simulink model "Task8_PWMSignal_2024b"  (R2025a)
settings: Solver=VariableStepAuto  StartTime=0.0  StopTime=10.0  RelTol=1e-3
libraries: simulink x2
settings Model: LastModifiedBy=Ashwin VJ

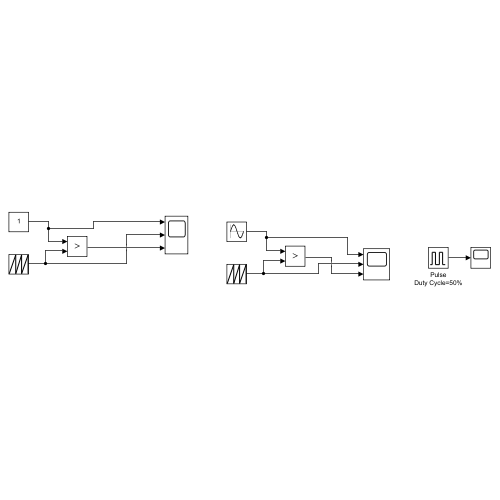
[thumbnail: Simulink's stored preview of the top-level diagram]
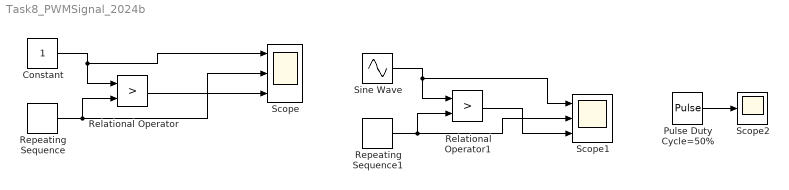
== system Task8_PWMSignal_2024b ==
  Constant : Constant
  Pulse Duty Cycle=50% : DiscretePulseGenerator  PulseType=Time based  PulseWidth=50
  Relational Operator : RelationalOperator  Operator=>  OutDataTypeStr=boolean  RndMeth=Simplest  InputSameDT=off
  Relational Operator1 : RelationalOperator  Operator=>  OutDataTypeStr=boolean  RndMeth=Simplest  InputSameDT=off
  Repeating Sequence : simulink/Sources/Repeating Sequence  rep_seq_t=[0 2]  rep_seq_y=[0 2]
  Repeating Sequence1 : simulink/Sources/Repeating Sequence  rep_seq_t=[0 2]  rep_seq_y=[0 2]
  Scope : Scope  NumInputPorts=3
      settings: ActiveDisplayYMinimum=0.9  ActiveDisplayYMaximum=1.1
  Scope1 : Scope  NumInputPorts=3
      settings: ActiveDisplayYMinimum=-1.2464592746769834  ActiveDisplayYMaximum=1.2491328116768927
  Scope2 : Scope
      settings: ActiveDisplayYMinimum=-0.12499999999999997  ActiveDisplayYMaximum=1.125  DataLoggingVariableName=ScopeData2
  Sine Wave : Sin  Frequency=2  SampleTime=0
  wires:
  Repeating Sequence/1 -> Scope/2, Relational Operator/2
  Constant/1 -> Scope/1, Relational Operator/1
  Relational Operator/1 -> Scope/3
  Repeating Sequence1/1 -> Scope1/2, Relational Operator1/2
  Relational Operator1/1 -> Scope1/3
  Sine Wave/1 -> Scope1/1, Relational Operator1/1
  Pulse Duty Cycle=50%/1 -> Scope2/1
